simulink model "openarm_system"  (R2026a)
settings: Solver=ode23t  StopTime=3  MaxStep=50e-6  RelTol=1e-4
values from neighbouring files (symbols this model uses):
  Pm = numeric_only(P)    [run_openarm.m]
  scen = struct('q0', wp(1,2:8)', 'v0', P.v_src - 0.3)    [run_openarm.m]
libraries: fl_lib x42, nesl_utility x24, robotmaniplib x6
settings Model: Creator=darsh  LastModifiedBy=darsh

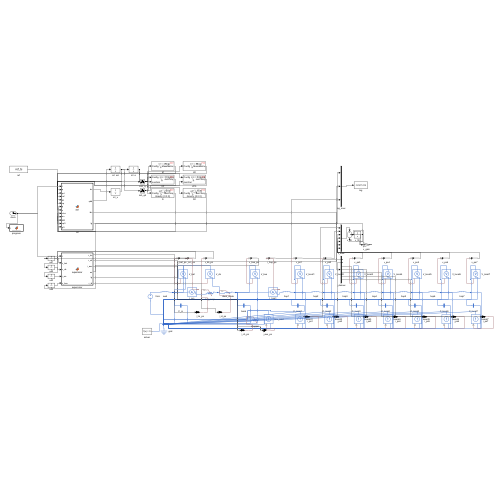
[thumbnail: Simulink's stored preview of the top-level diagram]
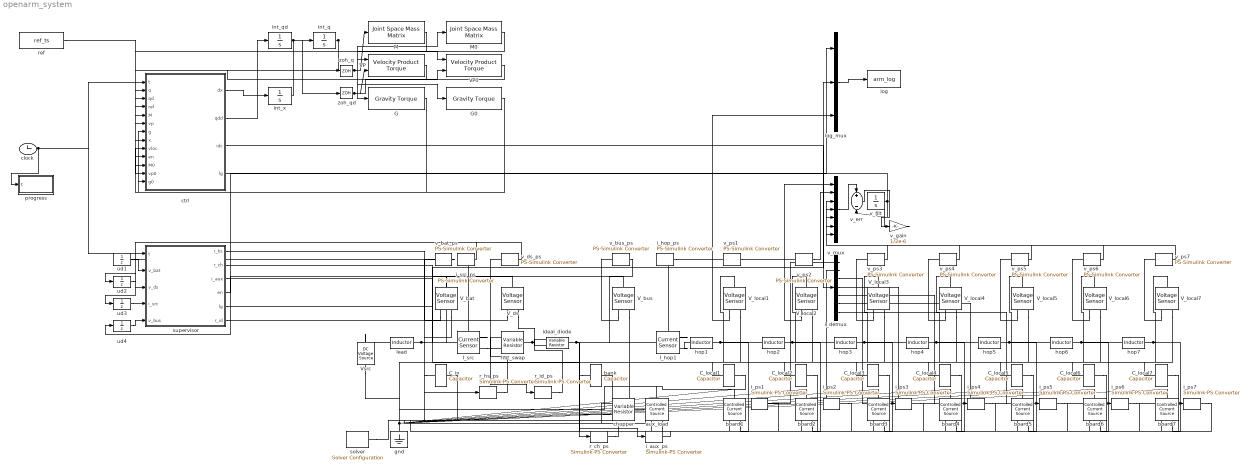
== system openarm_system ==
  C_in : fl_lib/Electrical/Electrical Elements/Capacitor  c=80e-6 F  r=0.05 Ohm  g=0 1/Ohm  i_specify=off  i_priority=None  i=0 A  i_nominal_specify=off  i_nominal_value=1  i_nominal_unit=A  v_specify=off  v_priority=None  v=0 V  v_nominal_specify=off  v_nominal_value=1  v_nominal_unit=V  vc_specify=on  vc_priority=High  vc=Pm.v_src V  vc_nominal_specify=off  vc_nominal_value=1  vc_nominal_unit=V
  C_local{1..7} (7 alike) : fl_lib/Electrical/Electrical Elements/Capacitor  c=Pm.c_local F  r=Pm.esr_local Ohm  g=0 1/Ohm  i_specify=off  i_priority=None  i=0 A  i_nominal_specify=off  i_nominal_value=1  i_nominal_unit=A  v_specify=off  v_priority=None  v=0 V  v_nominal_specify=off  v_nominal_value=1  v_nominal_unit=V  vc_specify=on  vc_priority=High  vc=scen.v0 V  vc_nominal_specify=off  vc_nominal_value=1  vc_nominal_unit=V
  G : robotmaniplib/Gravity Torque  RigidBodyTree=robot_sim  SimulateUsing=Code generation
  G0 : robotmaniplib/Gravity Torque  RigidBodyTree=robot_free  SimulateUsing=Code generation
  I_hop1 : fl_lib/Electrical/Electrical Sensors/Current Sensor
  I_src : fl_lib/Electrical/Electrical Sensors/Current Sensor
  M : robotmaniplib/Joint Space Mass Matrix  RigidBodyTree=robot_sim  SimulateUsing=Code generation
  M0 : robotmaniplib/Joint Space Mass Matrix  RigidBodyTree=robot_free  SimulateUsing=Code generation
  VP : robotmaniplib/Velocity Product Torque  RigidBodyTree=robot_sim  SimulateUsing=Code generation
  VP0 : robotmaniplib/Velocity Product Torque  RigidBodyTree=robot_free  SimulateUsing=Code generation
  V_bat : fl_lib/Electrical/Electrical Sensors/Voltage Sensor
  V_bus : fl_lib/Electrical/Electrical Sensors/Voltage Sensor
  V_ds : fl_lib/Electrical/Electrical Sensors/Voltage Sensor
  V_local{1..7} (7 alike) : fl_lib/Electrical/Electrical Sensors/Voltage Sensor
  Vsrc : fl_lib/Electrical/Electrical Sources/DC Voltage Source  v0=Pm.v_src V
  aux_load : fl_lib/Electrical/Electrical Sources/Controlled Current Source
  bank : fl_lib/Electrical/Electrical Elements/Capacitor  c=Pm.bank_c F  r=Pm.bank_esr Ohm  g=0 1/Ohm  i_specify=off  i_priority=None  i=0 A  i_nominal_specify=off  i_nominal_value=1  i_nominal_unit=A  v_specify=off  v_priority=None  v=0 V  v_nominal_specify=off  v_nominal_value=1  v_nominal_unit=V  vc_specify=on  vc_priority=High  vc=scen.v0 V  vc_nominal_specify=off  vc_nominal_value=1  vc_nominal_unit=V
  board{1..7} (7 alike) : fl_lib/Electrical/Electrical Sources/Controlled Current Source
  chopper : fl_lib/Electrical/Electrical Elements/Variable Resistor  Rmin=1e-3 Ohm  thermalEnable=false  thermal_mass=1 J/K  i_specify=off  i_priority=None  i=0 A  i_nominal_specify=off  i_nominal_value=1  i_nominal_unit=A  v_specify=off  v_priority=None  v=0 V  v_nominal_specify=off  v_nominal_value=1  v_nominal_unit=V  T_specify=off  T_priority=None  T=300 K  T_nominal_specify=off  T_nominal_value=1  T_nominal_unit=K
  clock : Clock
  ctrl : MATLAB Function  TreatAsAtomicUnit=on
  gnd : fl_lib/Electrical/Electrical Elements/Electrical Reference
  hop{1..7} (7 alike) : fl_lib/Electrical/Electrical Elements/Inductor  l=Pm.l_hop H  r=Pm.r_hop Ohm  g=1e-9 1/Ohm  i_specify=off  i_priority=None  i=0 A  i_nominal_specify=off  i_nominal_value=1  i_nominal_unit=A  v_specify=off  v_priority=None  v=0 V  v_nominal_specify=off  v_nominal_value=1  v_nominal_unit=V  i_L_specify=off  i_L_priority=High  i_L=0 A  i_L_nominal_specify=off  i_L_nominal_value=1  i_L_nominal_unit=A
  hot_swap : fl_lib/Electrical/Electrical Elements/Variable Resistor  Rmin=1e-5 Ohm  thermalEnable=false  thermal_mass=1 J/K  i_specify=off  i_priority=None  i=0 A  i_nominal_specify=off  i_nominal_value=1  i_nominal_unit=A  v_specify=off  v_priority=None  v=0 V  v_nominal_specify=off  v_nominal_value=1  v_nominal_unit=V  T_specify=off  T_priority=None  T=300 K  T_nominal_specify=off  T_nominal_value=1  T_nominal_unit=K
  i_aux_ps : nesl_utility/Simulink-PS Converter  PhysicalDomain=network_engine_domain  SubClassName=ps_input  LeftPortType=input  RightPortType=output  PseudoPeriodic=off  Frequencies=[]  NoiseDistribution=none  NoiseParameters=[]  Unit=1  AffineConversion=off  FilteringAndDerivatives=provide  SimscapeFilterOrder=1  InputFilterTimeConstant=0.001  UdotUserProvided=0
  i_demux : Demux  Outputs=7
  i_hop_ps : nesl_utility/PS-Simulink Converter  PhysicalDomain=network_engine_domain  SubClassName=ps_output  LeftPortType=input  RightPortType=output  PseudoPeriodic=off  Frequencies=[]  VectorFormat=inherit  Unit=inherit  AffineConversion=off
  i_ps{1..7} (7 alike) : nesl_utility/Simulink-PS Converter  PhysicalDomain=network_engine_domain  SubClassName=ps_input  LeftPortType=input  RightPortType=output  PseudoPeriodic=off  Frequencies=[]  NoiseDistribution=none  NoiseParameters=[]  Unit=1  AffineConversion=off  FilteringAndDerivatives=filter  SimscapeFilterOrder=1  InputFilterTimeConstant=5e-6  UdotUserProvided=0
  i_src_ps : nesl_utility/PS-Simulink Converter  PhysicalDomain=network_engine_domain  SubClassName=ps_output  LeftPortType=input  RightPortType=output  PseudoPeriodic=off  Frequencies=[]  VectorFormat=inherit  Unit=inherit  AffineConversion=off
  ideal_diode : fl_lib/Electrical/Electrical Elements/Variable Resistor  Rmin=1e-5 Ohm  thermalEnable=false  thermal_mass=1 J/K  i_specify=off  i_priority=None  i=0 A  i_nominal_specify=off  i_nominal_value=1  i_nominal_unit=A  v_specify=off  v_priority=None  v=0 V  v_nominal_specify=off  v_nominal_value=1  v_nominal_unit=V  T_specify=off  T_priority=None  T=300 K  T_nominal_specify=off  T_nominal_value=1  T_nominal_unit=K
  int_q : Integrator  InitialCondition=scen.q0
  int_qd : Integrator  InitialCondition=zeros(7,1)
  int_x : Integrator  InitialCondition=zeros(35,1)
  lead : fl_lib/Electrical/Electrical Elements/Inductor  l=Pm.l_lead H  r=Pm.r_lead + Pm.r_src Ohm  g=1e-9 1/Ohm  i_specify=off  i_priority=None  i=0 A  i_nominal_specify=off  i_nominal_value=1  i_nominal_unit=A  v_specify=off  v_priority=None  v=0 V  v_nominal_specify=off  v_nominal_value=1  v_nominal_unit=V  i_L_specify=off  i_L_priority=High  i_L=0 A  i_L_nominal_specify=off  i_L_nominal_value=1  i_L_nominal_unit=A
  log : ToWorkspace  VariableName=arm_log  SampleTime=Pm.Ts_log
  log_mux : Mux  Inputs=3
  progress : MATLAB Function  TreatAsAtomicUnit=on  SystemSampleTime=0.05
  r_ch_ps : nesl_utility/Simulink-PS Converter  PhysicalDomain=network_engine_domain  SubClassName=ps_input  LeftPortType=input  RightPortType=output  PseudoPeriodic=off  Frequencies=[]  NoiseDistribution=none  NoiseParameters=[]  Unit=1  AffineConversion=off  FilteringAndDerivatives=filter  SimscapeFilterOrder=1  InputFilterTimeConstant=20e-6  UdotUserProvided=0
  r_hs_ps : nesl_utility/Simulink-PS Converter  PhysicalDomain=network_engine_domain  SubClassName=ps_input  LeftPortType=input  RightPortType=output  PseudoPeriodic=off  Frequencies=[]  NoiseDistribution=none  NoiseParameters=[]  Unit=1  AffineConversion=off  FilteringAndDerivatives=filter  SimscapeFilterOrder=1  InputFilterTimeConstant=20e-6  UdotUserProvided=0
  r_id_ps : nesl_utility/Simulink-PS Converter  PhysicalDomain=network_engine_domain  SubClassName=ps_input  LeftPortType=input  RightPortType=output  PseudoPeriodic=off  Frequencies=[]  NoiseDistribution=none  NoiseParameters=[]  Unit=1  AffineConversion=off  FilteringAndDerivatives=filter  SimscapeFilterOrder=1  InputFilterTimeConstant=2e-6  UdotUserProvided=0
  ref : FromWorkspace  VariableName=ref_ts
  solver : nesl_utility/Solver Configuration  PhysicalDomain=network_engine_domain  SubClassName=solver  LeftPortType=input  RightPortType=generic  Tones=[]  Harmonics=[]  SimulateNoise=off  Profile=off  UseLocalSampling=off  EnableSwitchedLinearOptims=on  FrequencyDomain=off  UseCCode=off  RelTol=0.001  AbsTol=0.001  MinStep=1e-09  ToWorkspace=off  RevertToSquareIcSolve=off  NumHomotopyIterations=100  PhasorMode=off  PhasorModeNumHarmonics=1  ConsistencySolver=NEWTON_XTOL_AFTER_FTOL  CanonicalOrdering=CANONICAL  OptimizeIntermediates=OPTIMIZED  IndexReductionMethod=DerivativeReplacement  DoDC=off  ResidualTolerance=1e-09  ConsistencyTolSource=GLOBAL  ConsistencyAbsTol=0.001  ConsistencyRelTol=0.001  ConsistencyTolFactor=0.001  UseLocalSolver=off  LocalSolverChoice=NE_BACKWARD_EULER_ADVANCER  ResolveIndetEquations=on  FunctionEvalNumThread=1  LocalSolverSampleTime=0.001  DoFixedCost=off  MaxNonlinIter=3  MaxModeIter=2  ComputeImpulses=off  ImpulseIterations=2  LinearAlgebra=auto  LinearAlgebraNumThread=0  EquationFormulation=NE_TIME_EF  DelaysMemoryBudget=1024  AutomaticFiltering=on  FilteringTimeConstant=0.001  PartitionStorageMethod=AS_NEEDED  PartitionMemoryBudget=1024  PartitionMethod=ROBUST  MultibodyUseLocalSolver=off  MultibodyLocalSolverChoice=ODE1  MultibodyLocalSolverSampleTime=0.001
  supervisor : MATLAB Function  TreatAsAtomicUnit=on  SystemSampleTime=Pm.Ts_sup
  ud1 : UnitDelay  InitialCondition=scen.v0  SampleTime=Pm.Ts_sup
  ud2 : UnitDelay  SampleTime=Pm.Ts_sup
  ud3 : UnitDelay  SampleTime=Pm.Ts_sup
  ud4 : UnitDelay  InitialCondition=scen.v0  SampleTime=Pm.Ts_sup
  v_bat_ps : nesl_utility/PS-Simulink Converter  PhysicalDomain=network_engine_domain  SubClassName=ps_output  LeftPortType=input  RightPortType=output  PseudoPeriodic=off  Frequencies=[]  VectorFormat=inherit  Unit=inherit  AffineConversion=off
  v_bus_ps : nesl_utility/PS-Simulink Converter  PhysicalDomain=network_engine_domain  SubClassName=ps_output  LeftPortType=input  RightPortType=output  PseudoPeriodic=off  Frequencies=[]  VectorFormat=inherit  Unit=inherit  AffineConversion=off
  v_ds_ps : nesl_utility/PS-Simulink Converter  PhysicalDomain=network_engine_domain  SubClassName=ps_output  LeftPortType=input  RightPortType=output  PseudoPeriodic=off  Frequencies=[]  VectorFormat=inherit  Unit=inherit  AffineConversion=off
  v_err : Sum  Inputs=+-
  v_filt : Integrator  InitialCondition=scen.v0*ones(7,1)
  v_gain : Gain  Gain=1/2e-6
  v_mux : Mux  Inputs=7
  v_ps{1..7} (7 alike) : nesl_utility/PS-Simulink Converter  PhysicalDomain=network_engine_domain  SubClassName=ps_output  LeftPortType=input  RightPortType=output  PseudoPeriodic=off  Frequencies=[]  VectorFormat=inherit  Unit=inherit  AffineConversion=off
  zoh_q : ZeroOrderHold  SampleTime=Pm.Ts_dyn
  zoh_qd : ZeroOrderHold  SampleTime=Pm.Ts_dyn
  wires:
  v_ps1/1 -> v_mux/1
  i_demux/1 -> i_ps1/1
  v_ps2/1 -> v_mux/2
  i_demux/2 -> i_ps2/1
  v_ps3/1 -> v_mux/3
  i_demux/3 -> i_ps3/1
  v_ps4/1 -> v_mux/4
  i_demux/4 -> i_ps4/1
  v_ps5/1 -> v_mux/5
  i_demux/5 -> i_ps5/1
  v_ps6/1 -> v_mux/6
  i_demux/6 -> i_ps6/1
  v_ps7/1 -> v_mux/7
  i_demux/7 -> i_ps7/1
  clock/1 -> ctrl/1(t), supervisor/1(t), progress/1(t)
  int_q/1 -> ctrl/2(q), zoh_q/1
  int_qd/1 -> ctrl/3(qd), int_q/1, zoh_qd/1
  ref/1 -> ctrl/4(ref)
  M/1 -> ctrl/5(M)
  VP/1 -> ctrl/6(vp)
  G/1 -> ctrl/7(g)
  int_x/1 -> ctrl/8(x)
  M0/1 -> ctrl/11(M0)
  VP0/1 -> ctrl/12(vp0)
  G0/1 -> ctrl/13(g0)
  v_mux/1 -> v_err/1
  v_filt/1 -> v_err/2, ctrl/9(vloc)
  v_err/1 -> v_gain/1
  v_gain/1 -> v_filt/1
  ctrl/1(dx) -> int_x/1
  ctrl/2(qdd) -> int_qd/1
  ctrl/3(idc) -> i_demux/1
  zoh_q/1 -> M/1, VP/1, G/1, M0/1, VP0/1, G0/1
  zoh_qd/1 -> VP/2, VP0/2
  v_bat_ps/1 -> ud1/1
  ud1/1 -> supervisor/2(v_bat)
  v_ds_ps/1 -> ud2/1
  ud2/1 -> supervisor/3(v_ds)
  i_src_ps/1 -> ud3/1
  ud3/1 -> supervisor/4(i_src)
  v_bus_ps/1 -> ud4/1
  ud4/1 -> supervisor/5(v_bus)
  supervisor/1(r_hs) -> r_hs_ps/1
  supervisor/2(r_ch) -> r_ch_ps/1
  supervisor/3(i_aux) -> i_aux_ps/1
  supervisor/4(en) -> ctrl/10(en)
  supervisor/6(r_id) -> r_id_ps/1
  ctrl/4(lg) -> log_mux/1
  supervisor/5(lg) -> log_mux/2
  i_hop_ps/1 -> log_mux/3
  log_mux/1 -> log/1
  connections:
  solver/RConn1 -- Vsrc/RConn1 -- C_in/RConn1 -- V_bat/RConn2 -- bank/RConn1 -- V_bus/RConn2 -- chopper/RConn1 -- aux_load/LConn1 -- C_local1/RConn1 -- board1/LConn1 -- V_local1/RConn2 -- C_local2/RConn1 -- board2/LConn1 -- V_local2/RConn2 -- C_local3/RConn1 -- board3/LConn1 -- V_local3/RConn2 -- C_local4/RConn1 -- board4/LConn1 -- V_local4/RConn2 -- C_local5/RConn1 -- board5/LConn1 -- V_local5/RConn2 -- C_local6/RConn1 -- board6/LConn1 -- V_local6/RConn2 -- C_local7/RConn1 -- board7/LConn1 -- gnd/LConn1 -- V_local7/RConn2
  Vsrc/LConn1 -- lead/LConn1
  C_in/LConn1 -- lead/RConn1 -- I_src/LConn1 -- V_ds/LConn1 -- V_bat/LConn1
  I_src/RConn2 -- hot_swap/LConn2
  hot_swap/RConn1 -- V_ds/RConn2 -- ideal_diode/LConn2
  bank/LConn1 -- ideal_diode/RConn1 -- V_bus/LConn1 -- chopper/LConn2 -- aux_load/RConn2 -- I_hop1/LConn1
  I_hop1/RConn2 -- hop1/LConn1
  C_local1/LConn1 -- hop1/RConn1 -- board1/RConn2 -- V_local1/LConn1 -- hop2/LConn1
  V_local1/RConn1 -- v_ps1/LConn1
  i_ps1/RConn1 -- board1/RConn1
  C_local2/LConn1 -- hop2/RConn1 -- board2/RConn2 -- V_local2/LConn1 -- hop3/LConn1
  V_local2/RConn1 -- v_ps2/LConn1
  i_ps2/RConn1 -- board2/RConn1
  C_local3/LConn1 -- hop3/RConn1 -- board3/RConn2 -- V_local3/LConn1 -- hop4/LConn1
  V_local3/RConn1 -- v_ps3/LConn1
  i_ps3/RConn1 -- board3/RConn1
  C_local4/LConn1 -- hop4/RConn1 -- board4/RConn2 -- V_local4/LConn1 -- hop5/LConn1
  V_local4/RConn1 -- v_ps4/LConn1
  i_ps4/RConn1 -- board4/RConn1
  C_local5/LConn1 -- hop5/RConn1 -- board5/RConn2 -- V_local5/LConn1 -- hop6/LConn1
  V_local5/RConn1 -- v_ps5/LConn1
  i_ps5/RConn1 -- board5/RConn1
  C_local6/LConn1 -- hop6/RConn1 -- board6/RConn2 -- V_local6/LConn1 -- hop7/LConn1
  V_local6/RConn1 -- v_ps6/LConn1
  i_ps6/RConn1 -- board6/RConn1
  C_local7/LConn1 -- hop7/RConn1 -- board7/RConn2 -- V_local7/LConn1
  V_local7/RConn1 -- v_ps7/LConn1
  i_ps7/RConn1 -- board7/RConn1
  V_bat/RConn1 -- v_bat_ps/LConn1
  V_ds/RConn1 -- v_ds_ps/LConn1
  I_src/RConn1 -- i_src_ps/LConn1
  V_bus/RConn1 -- v_bus_ps/LConn1
  I_hop1/RConn1 -- i_hop_ps/LConn1
  r_hs_ps/RConn1 -- hot_swap/LConn1
  r_ch_ps/RConn1 -- chopper/LConn1
  i_aux_ps/RConn1 -- aux_load/RConn1
  r_id_ps/RConn1 -- ideal_diode/LConn1

== matlab function openarm_system/supervisor ==
  data: t input; r_hs output; v_bat input; v_ds input; i_src input; v_bus input; r_ch output; i_aux output; en output; lg output; r_id output; Pm parameter
function [r_hs, r_ch, i_aux, en, lg, r_id] = supervisor(t, v_bat, v_ds, i_src, v_bus, Pm)
% Support-board protection at Pm.Ts_sup (20 us): LM5069 hot-swap (current limit VCL/RS, power limit P/VDS, fault timer, LM5069-2
% retry at 0.5 % duty), primary chopper 57.1/55.0 V while the aux is alive, bus-powered backup 61.13/60.29 V with the
% TPS3700 delays, aux load, the actuator drive-enable used by the scenarios, and the LTC4359 ideal diode: on with
% r_id once its input (BAT+ less the hot-swap drop) exceeds the bus by its 30 mV forward-regulation voltage, off (fast pull-down, < 0.5 us) once the bus
% exceeds that input by 30 mV (LTC4359 Rev. F: dVSD 30 mV regulation, FPD comparator, tOFF 0.3-0.5 us).
persistent rlim tmr off_until pri bak bak_pend bak_t idon
if isempty(rlim)
    rlim = 0; tmr = 0; off_until = -1; pri = 0; bak = 0; bak_pend = 0; bak_t = 0; idon = 1;
end
Ts = Pm.Ts_sup;
aux = double(t < Pm.t_aux_fail);
% hot-swap
i_eff = min(Pm.i_lim, Pm.p_lim/max(v_ds, 0.5));
if t < off_until
    r_hs = 1e4; rlim = 0;
else
    rlim = max(0, rlim + Ts*Pm.k_lim*(i_src - i_eff));
    if rlim > 1e-4
        tmr = tmr + Ts;
    else
        tmr = max(0, tmr - Ts*2.5/85);
    end
    if tmr >= Pm.t_flt
        off_until = t + Pm.t_flt/Pm.retry_duty; tmr = 0; rlim = 0;
    end
    r_hs = Pm.r_hs + rlim;
    if t < off_until
        r_hs = 1e4;
    end
end
% chopper: primary needs the aux; backup needs only the bus
if aux > 0 && Pm.pri_en > 0
    if v_bus > Pm.chop_pri(1), pri = 1; elseif v_bus < Pm.chop_pri(2), pri = 0; end
else
    pri = 0;
end
want = bak;
if Pm.backup > 0
    if v_bus > Pm.chop_bak(1), want = 1; elseif v_bus < Pm.chop_bak(2), want = 0; end
else
    want = 0;
end
if want ~= bak
    if bak_pend == 0
        bak_pend = 1; bak_t = t + Pm.t_bak(2 - want);
    elseif t >= bak_t
        bak = want; bak_pend = 0;
    end
else
    bak_pend = 0;
end
on = max(pri, bak);
r_ch = on*Pm.r_brake + (1 - on)*1e4;
i_aux = aux*Pm.p_aux/max(v_bus, 10);
en = double(t < Pm.t_drv_off);
v_in = v_bat - v_ds;                                         % LTC4359 IN = hot-swap output
% fix 5 Nov 2026: LTC4359 blocks reverse current (off once OUT > IN), back on at 30 mV forward; 30 mV hysteresis kept
if v_bus > v_in, idon = 0; elseif v_in - v_bus > 0.03, idon = 1; end
r_id = idon*Pm.r_id + (1 - idon)*1e4;
lg = [v_bat; v_bus; i_src; v_ds; r_hs; on; pri; bak; aux; double(t < off_until)];
end

== matlab function openarm_system/ctrl ==
  data: t input; dx output; q input; qd input; ref input; M input; vp input; g input; x input; vloc input; en input; M0 input; vp0 input; g0 input; qdd output; idc output; lg output; Pm parameter
function [dx, qdd, idc, lg] = ctrl(t, q, qd, ref, M, vp, g, x, vloc, en, M0, vp0, g0, Pm)
% Joint control, averaged FOC actuators and arm acceleration for openarm_system.slx (all vectors are joint 1..7).
% Computed-torque PID position loop -> iq command -> dq PI current loops with back-EMF feedforward and the SVPWM voltage
% limit set by each board's local bus -> torque through gear efficiency (eta motoring, 1/eta generating) and friction
% -> qdd = (M + J_refl) \ (tau - vp - g). DC current per board = (dq power + conduction + switching + board) / V.
% M, vp, g include the payload and are what the controller uses throughout; M0, vp0, g0 are the arm without it. The plant
% switches to them at Pm.t_release (the controller is not told). en = 0 is gates off (safe torque off): each inverter is
% a diode bridge, so the motor drives current into its board's bus only when the back-EMF exceeds vloc / sqrt(3).
% Joint hard stops 2 deg outside the URDF limits: spring Pm.k_stop and damper Pm.c_stop while in contact.
N = Pm.N(:); kt = Pm.kt_m(:); eta = Pm.eta(:); L = Pm.L(:); R = Pm.R(:); lam = Pm.lambda(:); pp = Pm.pp(:);
id = x(1:7); iq = x(8:14); zd = x(15:21); zq = x(22:28); ze = x(29:35);
qr = ref(1:7); qdr = ref(8:14); qddr = ref(15:21);
Mt = M + diag(Pm.J_refl(:));
fric = Pm.tau_coulomb(:).*tanh(qd/0.01) + Pm.b_visc(:).*qd;
a = qddr + Pm.kp_q(:).*(qr - q) + Pm.kd_q(:).*(qdr - qd) + Pm.ki_q(:).*ze;
tau_cmd = Mt*a + vp + g + fric;
tau_cmd = min(max(tau_cmd, -Pm.tau_max(:)), Pm.tau_max(:));
iq_ref = en*tau_cmd./(N.*kt*Pm.eta_hat);       % controller assumes one nominal efficiency
iq_ref = min(max(iq_ref, -Pm.i_max(:)), Pm.i_max(:));
wm = N.*qd; we = pp.*wm;
ed = -id; eq = iq_ref - iq;
vd = Pm.kp_i(:).*ed + zd - we.*L.*iq;
vq = Pm.kp_i(:).*eq + zq + we.*lam + we.*L.*id;
vmax = Pm.v_frac*max(vloc, 0);
vm = sqrt(vd.^2 + vq.^2);
s = min(1, vmax./max(vm, 1e-9));
vd = vd.*s; vq = vq.*s;
free = double(s >= 0.999);
if en < 0.5
    imag0 = sqrt(id.^2 + iq.^2 + Pm.i_eps^2);
    vdi = max(vloc, 0)/sqrt(3);
    vd = -vdi.*id./imag0; vq = -vdi.*iq./imag0;
end
dzd = en*Pm.ki_i(:).*ed.*free - (1-en)*zd*1e3;
dzq = en*Pm.ki_i(:).*eq.*free - (1-en)*zq*1e3;
did = (vd - R.*id + we.*L.*iq)./L;
diq = (vq - R.*iq - we.*L.*id - we.*lam)./L;
tm = kt.*iq;
pm = tm.*wm;
eff = eta.^tanh(pm/2);
tau = N.*tm.*eff - fric;
pen = max(q - Pm.q_hi(:), 0) + min(q - Pm.q_lo(:), 0);
tau = tau - Pm.k_stop*pen - Pm.c_stop*qd.*min(1, abs(pen)/1e-3);
pl = double(t < Pm.t_release);
Mp = pl*Mt + (1 - pl)*(M0 + diag(Pm.J_refl(:)));
qdd = Mp \ (tau - pl*(vp + g) - (1 - pl)*(vp0 + g0));
imag = sqrt(id.^2 + iq.^2);
pe = 1.5*(vd.*id + vq.*iq);
pdc = pe + 1.5*imag.^2*Pm.rds + en*3*vloc.*imag*(2/pi)*Pm.t_sw*Pm.fsw + Pm.p_board;
idc = pdc./max(vloc, 10);
dx = [did; diq; dzd; dzq; en*(qr - q)];
lg = [t; q; qd; qr; iq; iq_ref; tau; pdc; vloc];
end

== matlab function openarm_system/progress ==
  data: t input
function progress(t)
fprintf('t = %.2f s\n', t);
end
